simulink model "ZT_VehCtrl_18B_CAN"  (R2018b)
settings: Solver=FixedStepAuto  StartTime=0.0  StopTime=inf  FixedStep=0.005  RelTol=1e-3
InitFcn:
  | mbd_mpc_consistency_checks(bdroot(gcs));
values from neighbouring files (symbols this model uses):
  BatoverTempTh = single(80)    [VCU_INIT.m]
  BRS_PwrValid = single(5)    [VCU_INIT.m]
  BRSEnSpdTh1 = single(10)    [VCU_INIT.m]
  BRSEnSpdTh2 = single(20)    [VCU_INIT.m]
  MCUTempAlarmTh = single (60)    [VCU_INIT.m]
  mps2kmh = single(3.6)    [VCU_INIT.m]
  MtrPwrFac = single(1/9550)    [VCU_INIT.m]
  MtrTempAlarmTh = single (50)    [VCU_INIT.m]
  Padle1Signal1_Th = [PadleSignal1_min,PadleSignal1_max]    [VCU_INIT.m]
  Padle1Signal2_Th = [PadleSignal2_min,PadleSignal2_max]    [VCU_INIT.m]
  PadleSignal1_max = 3.84    [VCU_INIT.m]
  PadleSignal1_min = 0.75    [VCU_INIT.m]
  PadleSignal2_max = 1.92    [VCU_INIT.m]
  PadleSignal2_min = 0.375    [VCU_INIT.m]
  PadleValid = 0.05    [VCU_INIT.m]
  PwrLimFactor = single(0.5)    [VCU_INIT.m]
  Ratio = single(1)    [VCU_INIT.m]
  rpm2mps = single(2*pi/60 * WhlRadius/Ratio)    [VCU_INIT.m]
  SOCLowTh = single(20)    [VCU_INIT.m]
  VehPwrBackwardMax = VehPwrMax * single(0.3)    [VCU_INIT.m]
  VehPwrMax = single(MtrPwrMax * 4)    [VCU_INIT.m]
  VehTrqBackwardMax = VehTrqMax * single(0.3)    [VCU_INIT.m]
  VehTrqMax = single(MtrTrqMax * Ratio *4)    [VCU_INIT.m]
  WhlRadius = single(1)    [VCU_INIT.m]
undefined symbols (not defined in the file or in its folder): Delay_Charge, Delay_Discharge, fifo_0_vect, fifo_1_vect, LQFP, pts1_fifo_0_vect, pts1_fifo_1_vect, pts2_fifo_0_vect, pts2_fifo_1_vect, pts3_fifo_0_vect, pts3_fifo_1_vect, pts4_fifo_0_vect, pts4_fifo_1_vect
libraries: mbd_mpc574x_ec_toolbox x157, canmsglib x74, simulink x38
(part 12 of 12)

== system ZT_VehCtrl_18B_CAN/SigOut/GPIO /SPI3: LS03_06_07_08_10_12_13_17_18_19/Subsystem/控制 ==
  note: out1
  note: out2
  note: out3
  note: out5
  note: out4
  note: out7
  note: out6
  note: out8
  Add : Sum  Inputs=++++++++
  Add1 : Sum  Inputs=+++
  Constant1 : Constant  Value=0
  Constant2 : Constant  Value=0
  Constant9 : Constant  Value=44  OutDataTypeStr=uint8
  Data Store Read : DataStoreRead  DataStoreName=LS019
  Data Store Read1 : DataStoreRead  DataStoreName=LS007
  Data Store Read10 : DataStoreRead  DataStoreName=LS006
  Data Store Read2 : DataStoreRead  DataStoreName=LS012
  Data Store Read4 : DataStoreRead  DataStoreName=LS018
  Data Store Read5 : DataStoreRead  DataStoreName=LS010
  Data Store Read6 : DataStoreRead  DataStoreName=LS008
  Data Store Read7 : DataStoreRead  DataStoreName=LS003
  Data Store Read8 : DataStoreRead  DataStoreName=LS017
  Data Store Read9 : DataStoreRead  DataStoreName=LS013
  Data Type Conversion : DataTypeConversion  OutDataTypeStr=uint8
  Data Type Conversion1 : DataTypeConversion  OutDataTypeStr=uint8
  Gain : Gain
  Gain1 : Gain  Gain=2
  Gain2 : Gain  Gain=4
  Gain3 : Gain  Gain=8
  Gain4 : Gain  Gain=16
  Gain5 : Gain  Gain=32
  Gain6 : Gain  Gain=64
  Gain7 : Gain  Gain=128
  Gain8 : Gain
  Gain9 : Gain  Gain=2
  Terminator{,1..3} (4 alike) : Terminator
  Out1 : Outport  VectorParamsAs1DForOutWhenUnconnected=on
  Out2 : Outport  Port=2  VectorParamsAs1DForOutWhenUnconnected=on
  wires:
  Constant9/1 -> Add1/1
  Data Store Read10/1 -> Gain7/1
  Data Type Conversion1/1 -> Out2/1
  Data Store Read2/1 -> Gain9/1
  Add1/1 -> Data Type Conversion/1
  Add/1 -> Data Type Conversion1/1
  Data Store Read5/1 -> Gain2/1
  Gain6/1 -> Add/2
  Data Store Read1/1 -> Gain8/1
  Gain9/1 -> Add1/2
  Gain7/1 -> Add/1
  Gain/1 -> Add/8
  Data Type Conversion/1 -> Out1/1
  Data Store Read9/1 -> Gain6/1
  Gain4/1 -> Add/4
  Gain8/1 -> Add1/3
  Gain1/1 -> Add/7
  Data Store Read6/1 -> Gain3/1
  Gain3/1 -> Add/5
  Gain2/1 -> Add/6
  Gain5/1 -> Add/3
  Data Store Read8/1 -> Terminator/1
  Data Store Read7/1 -> Terminator1/1
  Constant1/1 -> Gain4/1, Gain5/1
  Data Store Read/1 -> Terminator3/1
  Data Store Read4/1 -> Terminator2/1
  Constant2/1 -> Gain/1, Gain1/1

== stateflow chart ZT_VehCtrl_18B_CAN/VehCtrl/EnergyManage/Chart ==
  state Charging
    en:
    Ready = false;
    VCU_PowerOnReq = 0;
    VCU_UrgencyCutOffPowerReq = 0 ;
    VCU_DCDC1_En = 1;
    DcdcCmd = 1;
    DcacEpsCmd = 1;
    VCU2OilMotor_ActiveDisCharge = 0;
    VCU2DrvMotor_ActiveDisCharge = 0;
    TM_Discharge = 0;
    ISG_Discharge = 0;
    EDrv1_PowOnCmd = 0;
    EDrv2_PowOnCmd = 0;
    VCU_ShrRlyCtl = 0;
    VCU_HghVtgCtl = 0;
    VCU_DCCpstRlyCtl = 1;
    Flag = 6;
  state Init
    en:
    Ready = false;
    VCU_PowerOnReq = 0;
    VCU_UrgencyCutOffPowerReq = 0 ;
    VCU_DCDC1_En = 0;
    DcdcCmd = 0;
    DcacEpsCmd = 0;
    VCU2OilMotor_ActiveDisCharge = 0;
    VCU2DrvMotor_ActiveDisCharge = 0;
    TM_Discharge = 0;
    ISG_Discharge = 0;
    EDrv1_PowOnCmd = 0;
    EDrv2_PowOnCmd = 0;
    VCU_ShrRlyCtl = 0;
    VCU_HghVtgCtl = 0;
    VCU_DCCpstRlyCtl = 0;
    OnOffCmd = 0;
    Flag = 1;
  state EmgencyDown
    Ready = false;
    VCU_PowerOnReq = 0;
    VCU_UrgencyCutOffPowerReq = 1 ;
    VCU_DCDC1_En = 2;
    DcdcCmd = 0
    DcacEpsCmd = 0;
    VCU2DrvMotor_En = 0 ;
    VCU2OilMotor_ActiveDisCharge = 1;
    VCU2DrvMotor_ActiveDisCharge = 1;
    TM_Discharge = 1;
    ISG_Discharge = 1;
    EDrv1_PowOnCmd = 0;
    EDrv2_PowOnCmd = 0;
    VCU_ShrRlyCtl = 0;
    VCU_HghVtgCtl = 0;
    Flag = 5;
    du:OnOffCmd = 0;
  state PowerDown
    Ready = false;
    VCU_PowerOnReq = 0;
    VCU_UrgencyCutOffPowerReq = 0;
    VCU_DCDC1_En = 2;
    DcdcCmd = 0
    DcacEpsCmd = 0;
    VCU2OilMotor_ActiveDisCharge = 1;
    VCU2DrvMotor_ActiveDisCharge = 1;
    TM_Discharge = 1;
    ISG_Discharge = 1;
    EDrv1_PowOnCmd = 0;
    EDrv2_PowOnCmd = 0;
    VCU_ShrRlyCtl = 0;
    VCU_HghVtgCtl = 0;
    Flag = 4;
    du:OnOffCmd = 0;
  state PowerOn
    state Hv_Req
      Ready = false;
      VCU_PowerOnReq = 1;
      VCU_HghVtgCtl = 1;
      Flag = 2；
    state Ready
      en:
      Ready = true;
      VCU_PowerOnReq = 1;
      VCU_UrgencyCutOffPowerReq = 0 ;
      VCU_DCDC1_En = 1;
      DcdcCmd = 1
      DcacEpsCmd = 1;
      VCU2OilMotor_ActiveDisCharge = 0;
      VCU2DrvMotor_ActiveDisCharge = 0;
      TM_Discharge = 0;
      ISG_Discharge = 0;
      EDrv1_PowOnCmd = 1;
      EDrv2_PowOnCmd = 1;
      VCU_ShrRlyCtl = 1;
      VCU_HghVtgCnt = 1;
      Flag = 3;
      du:OnOffCmd = 0;
    (default) -> Hv_Req
    Hv_Req -> Ready : [BMS_PrechargeStatus == 2&&BMS_ReadySt == 1]
  state EnBRS
    en:
    BRS_PowerReq = PwrCupReq-BMS_ChgPwrMax;
    MaxChargePowerLimit = BMS_ChgPwrMax;
    Flag = 7
    du:OnOffCmd = 1;
  Charging -> Init : [ChargeSig == 0&&Cnt>Delay_Charge]
  Init -> Charging [order 2] : [ChargeSig == 1&&NonOBC == 0]{Cnt = 0;}
  EmgencyDown -> Init : [Cnt>Delay_Discharge&&BMS_ReadySt == 0]
  (default) -> Init
  PowerDown -> Init : [Cnt>Delay_Discharge&&BMS_ReadySt == 0]
  Init -> PowerOn [order 1] : [Key == 1&&ShutDown == 0]
  PowerOn -> PowerDown [order 2] : [Key == 0&&ShutDown == 0]{Cnt = 0;}
  PowerOn -> EmgencyDown [order 1] : [ShutDown>0]{Cnt = 0;}
  EnBRS -> Ready : [AccPadle >0.1||VehSpdFb<BRSEnSpdTh1]
  Ready -> EnBRS : [AccPadle <0.05&&VehSpdFb>BRSEnSpdTh2&&NonBRS == 0]
  data: VCU_PowerOnReq output; VCU_UrgencyCutOffPowerReq output; VCU_DCDC1_En output; MaxChargePowerLimit output; BRS_PowerReq output; OnOffCmd output; EDrv1_PowOnCmd output; EDrv2_PowOnCmd output; VCU2OilMotor_ActiveDisCharge output; VCU2DrvMotor_ActiveDisCharge output; DcdcCmd output; DcacEpsCmd output; VCU_ShrRlyCtl output; VCU_HghVtgCtl output; VCU_DCCpstRlyCtl output; BMS_ReadySt input; BMS_PrechargeStatus input; BMS_BatteryPower input; OBC_Start input; Ready output; Flag output; Key input; Cnt local; Delay_Discharge parameter single; Delay_Charge parameter; PwrCupReq input; BMS_ChgPwrMax input; BRS_PwrValid parameter; ShutDown input; NonBRS input; NonOBC input; ChargeSig input; TM_Discharge output; ISG_Discharge output; AccPadle input; VehSpdFb input; BRSEnSpdTh1 parameter double; BRSEnSpdTh2 parameter

== stateflow chart ZT_VehCtrl_18B_CAN/SigOut/GPIO /PWM_OUT/FreqCMD ==
  settings: executeAtInitialization=1
  state A
    du:
    freq = 20000;
    cntr = cntr + 1;
    dc = 0.25;
  state A1
    du:
    freq = 10000;
    cntr = cntr - 1;
    dc =  0.5;
  (default) -> A : {cntr=0;dc=0;}
  A1 -> A : [cntr < 1]
  A -> A1 : [cntr > 50]
  data: cntr local uint32 =0; freq output uint32; dc output single

== stateflow chart ZT_VehCtrl_18B_CAN/Initialization & SPI timer1/CS1 LS/Chart ==
  state clear
    en:high=128+7;low=1;cnt=0;
    du:cnt = cnt + 1;
  state en
    en:high=128+1+64;low=0;cnt=0;
    du:cnt = cnt + 1;
  state config
    en:high=128+7+64;low=1+128;cnt=0;
    du:cnt = cnt + 1;
  (default) -> clear
  clear -> en : [cnt>5]
  en -> config : [cnt>5]
  data: high output; low output; cnt local

== stateflow chart ZT_VehCtrl_18B_CAN/Initialization & SPI timer1/CS3 LS/Chart ==
  state ConfigA
    en:high=80+mode*(1+4);low=0+mode*(1+4);cnt=0;
    du:cnt = cnt + 1;
  state en
    en:high=96;low=0;cnt=0;
  (default) -> ConfigA
  ConfigA -> en : [cnt>4]
  data: high output; low output; cnt local; mode input

== stateflow chart ZT_VehCtrl_18B_CAN/Initialization & SPI timer1/CS5 LS/Chart ==
  state clear
    en:high=128+7;low=1;cnt=0;
    du:cnt = cnt + 1;
  state en
    en:high=128+1+64;low=0;cnt=0;
    du:cnt = cnt + 1;
  state config
    en:high=128+7+64;low=1+128;cnt=0;
  (default) -> clear
  clear -> en : [cnt>5]
  en -> config : [cnt>5]
  data: high output; low output; cnt local

== stateflow chart ZT_VehCtrl_18B_CAN/Initialization & SPI timer1/Chart ==
  state Idle
    en:Flg=0;
  state Initialize
    en:Flg=1;
  state Normal
    en:Flg=2;
  (default) -> Idle
  Normal -> Idle : [ResetFlg==1]
  Initialize -> Idle [order 2] : [ResetFlg==1]
  Idle -> Initialize : [ResetFlg==0]
  Initialize -> Normal [order 1] : [InitFlg>0]
  data: ResetFlg input; InitFlg input; Flg output

== stateflow chart ZT_VehCtrl_18B_CAN/Initialization & SPI timer1/Chart1 ==
  state IDLE
    en:Flg=0;
  state CS1
    en:Flg=1;cnt=0;
    du:cnt = cnt + 1;
  state CS5
    en:Flg=2;cnt=0;
    du:cnt = cnt + 1;
  state Done
    en:Flg=9;
  (default) -> IDLE
  Done -> IDLE : [VcuMode==0]
  IDLE -> CS1 : [VcuMode==1]
  CS1 -> CS5 : [cnt>20]
  CS5 -> Done : [cnt>20]
  data: VcuMode input; Flg output; cnt local

== stateflow chart ZT_VehCtrl_18B_CAN/Initialization & SPI timer1/Chart2 ==
  state IDLE
    en:Flg=0;
  state CS2
    en:Flg=1;cnt=0;
    du:cnt = cnt + 1;
  state CS3
    en:Flg=2;cnt=0;
    du:cnt = cnt + 1;
  state Done
    en:Flg=9;
  (default) -> IDLE
  Done -> IDLE : [VcuMode==0]
  IDLE -> CS2 : [VcuMode==1]
  CS2 -> CS3 : [cnt>20]
  CS3 -> Done : [cnt>20]
  data: VcuMode input; Flg output; cnt local
